simulink model "AXU5EV_Motor_Control_System"  (R2026b)
settings: Solver=FixedStepDiscrete  StopTime=0.1
model workspace (MAT data in the model file):
  ADC_Calibration_Log2_N = 10
  ADC_Manual_Offset_Valid_A = 0
  ADC_Manual_Offset_Valid_B = 0
  Angle_Init_EN = Simulink.Signal
  Angle_Init_EN.InitialValue = '0'
  Angle_Init_EN.DataType = 'double'
  Encoder_Counts_Per_Electrical_Period = 30000
  Encoder_Nanometres_Per_Count = 1000
  Experiment_Id_Limit_A = 0.5
  Experiment_Iq_Limit_A = 0.3
  Experiment_Parameter_Version = 20261117
  FOC_Fixed_Config.Version = 20261024
  FOC_Fixed_Config.Parameters.Rs = 1.45
  FOC_Fixed_Config.Parameters.Ld = 0.0118
  FOC_Fixed_Config.Parameters.Lq = 0.0118
  FOC_Fixed_Config.Parameters.psi = 0.0684240400279
  FOC_Fixed_Config.Parameters.Kp_ACR = 59
  FOC_Fixed_Config.Parameters.Ki_ACR = 7250
  FOC_Fixed_Config.Parameters.Kaw_d = 0.0122881355932
  FOC_Fixed_Config.Parameters.Kaw_q = 0.0122881355932
  FOC_Fixed_Config.Parameters.Ts_ACR = 0.0001
  FOC_Fixed_Config.Parameters.Udc = 48
  FOC_Fixed_Config.Fimath = embedded.fimath
  FOC_Fixed_Config.Fimath.RoundMode = 'convergent'
  FOC_Fixed_Config.Fimath.RoundingMethod = 'Convergent'
  FOC_Fixed_Config.Fimath.OverflowMode = 'saturate'
  FOC_Fixed_Config.Fimath.OverflowAction = 'Saturate'
  FOC_Fixed_Config.Fimath.ProductMode = 'FullPrecision'
  FOC_Fixed_Config.Fimath.SumMode = 'FullPrecision'
  FOC_Fixed_Config.Fimath.FixedOpFloatingYields = 'Fixed'
  FOC_Fixed_Config.Fimath.ProductWordLength = 32
  FOC_Fixed_Config.Fimath.SumWordLength = 32
  FOC_Fixed_Config.Fimath.MaxProductWordLength = 65535
  FOC_Fixed_Config.Fimath.MaxSumWordLength = 65535
  FOC_Fixed_Config.Fimath.ProductFractionLength = 30
  FOC_Fixed_Config.Fimath.ProductFixedExponent = -30
  FOC_Fixed_Config.Fimath.SumFractionLength = 30
  FOC_Fixed_Config.Fimath.SumFixedExponent = -30
  FOC_Fixed_Config.Fimath.SumSlopeAdjustmentFactor = 1
  FOC_Fixed_Config.Fimath.SumBias = 0
  FOC_Fixed_Config.Fimath.ProductSlopeAdjustmentFactor = 1
  FOC_Fixed_Config.Fimath.ProductBias = 0
  FOC_Fixed_Config.Fimath.CastBeforeSum = 1
  FOC_Fixed_Config.Fimath.SumSlope = 9.31322574615e-10
  FOC_Fixed_Config.Fimath.ProductSlope = 9.31322574615e-10
  FOC_Fixed_Config.Fimath.DDGMaxProductWordLength = 65535
  FOC_Fixed_Config.Fimath.DDGMaxSumWordLength = 65535
  FOC_Fixed_Config.Fimath.DDGProductFixedExponent = -30
  FOC_Fixed_Config.Fimath.DDGProductFractionLength = 30
  FOC_Fixed_Config.Fimath.DDGProductWordLength = 32
  FOC_Fixed_Config.Fimath.DDGSumFixedExponent = -30
  FOC_Fixed_Config.Fimath.DDGSumFractionLength = 30
  FOC_Fixed_Config.Fimath.DDGSumWordLength = 32
  FOC_Fixed_Config.Fimath.DDGProductBias = 0
  FOC_Fixed_Config.Fimath.DDGProductSlopeAdjustmentFactor = 1
  FOC_Fixed_Config.Fimath.DDGSumBias = 0
  FOC_Fixed_Config.Fimath.DDGSumSlopeAdjustmentFactor = 1
  FOC_Fixed_Config.Fimath.DDGCastBeforeSum = 1
  FOC_Fixed_Config.Fimath.DDGProductSlope = 9.31322574615e-10
  FOC_Fixed_Config.Fimath.DDGSumSlope = 9.31322574615e-10
  FOC_Fixed_Config.Types.Current = embedded.numerictype
  FOC_Fixed_Config.Types.Current.ReadOnly = 0
  FOC_Fixed_Config.Types.Current.Volatile = 0
  FOC_Fixed_Config.Types.Current.DataTypeMode = 'Fixed-point: binary point scaling'
  FOC_Fixed_Config.Types.Current.DataType = 'Fixed'
  FOC_Fixed_Config.Types.Current.Scaling = 'BinaryPoint'
  FOC_Fixed_Config.Types.Current.SignednessBool = 1
  FOC_Fixed_Config.Types.Current.Signedness = 'Signed'
  FOC_Fixed_Config.Types.Current.Signed = 1
  FOC_Fixed_Config.Types.Current.WordLength = 32
  FOC_Fixed_Config.Types.Current.FractionLength = 24
  FOC_Fixed_Config.Types.Current.BinaryPoint = 24
  FOC_Fixed_Config.Types.Current.Slope = 5.96046447754e-08
  FOC_Fixed_Config.Types.Current.FixedExponent = -24
  FOC_Fixed_Config.Types.Current.SlopeAdjustmentFactor = 1
  FOC_Fixed_Config.Types.Current.Bias = 0
  FOC_Fixed_Config.Types.Current.DataTypeOverride = 'Inherit'
  FOC_Fixed_Config.Types.Angle = embedded.numerictype
  FOC_Fixed_Config.Types.Angle.ReadOnly = 0
  FOC_Fixed_Config.Types.Angle.Volatile = 0
  FOC_Fixed_Config.Types.Angle.DataTypeMode = 'Fixed-point: binary point scaling'
  FOC_Fixed_Config.Types.Angle.DataType = 'Fixed'
  FOC_Fixed_Config.Types.Angle.Scaling = 'BinaryPoint'
  FOC_Fixed_Config.Types.Angle.SignednessBool = 1
  FOC_Fixed_Config.Types.Angle.Signedness = 'Signed'
  FOC_Fixed_Config.Types.Angle.Signed = 1
  FOC_Fixed_Config.Types.Angle.WordLength = 40
  FOC_Fixed_Config.Types.Angle.FractionLength = 32
  FOC_Fixed_Config.Types.Angle.BinaryPoint = 32
  FOC_Fixed_Config.Types.Angle.Slope = 2.32830643654e-10
  FOC_Fixed_Config.Types.Angle.FixedExponent = -32
  FOC_Fixed_Config.Types.Angle.SlopeAdjustmentFactor = 1
  FOC_Fixed_Config.Types.Angle.Bias = 0
  FOC_Fixed_Config.Types.Angle.DataTypeOverride = 'Inherit'
  FOC_Fixed_Config.Types.Omega = embedded.numerictype
  FOC_Fixed_Config.Types.Omega.ReadOnly = 0
  FOC_Fixed_Config.Types.Omega.Volatile = 0
  FOC_Fixed_Config.Types.Omega.DataTypeMode = 'Fixed-point: binary point scaling'
  FOC_Fixed_Config.Types.Omega.DataType = 'Fixed'
  FOC_Fixed_Config.Types.Omega.Scaling = 'BinaryPoint'
  FOC_Fixed_Config.Types.Omega.SignednessBool = 1
  FOC_Fixed_Config.Types.Omega.Signedness = 'Signed'
  FOC_Fixed_Config.Types.Omega.Signed = 1
  FOC_Fixed_Config.Types.Omega.WordLength = 40
  FOC_Fixed_Config.Types.Omega.FractionLength = 24
  FOC_Fixed_Config.Types.Omega.BinaryPoint = 24
  FOC_Fixed_Config.Types.Omega.Slope = 5.96046447754e-08
  FOC_Fixed_Config.Types.Omega.FixedExponent = -24
  FOC_Fixed_Config.Types.Omega.SlopeAdjustmentFactor = 1
  FOC_Fixed_Config.Types.Omega.Bias = 0
  FOC_Fixed_Config.Types.Omega.DataTypeOverride = 'Inherit'
  FOC_Fixed_Config.Types.Bus = embedded.numerictype
  FOC_Fixed_Config.Types.Bus.ReadOnly = 0
  FOC_Fixed_Config.Types.Bus.Volatile = 0
  FOC_Fixed_Config.Types.Bus.DataTypeMode = 'Fixed-point: binary point scaling'
  FOC_Fixed_Config.Types.Bus.DataType = 'Fixed'
  FOC_Fixed_Config.Types.Bus.Scaling = 'BinaryPoint'
  FOC_Fixed_Config.Types.Bus.SignednessBool = 0
  FOC_Fixed_Config.Types.Bus.Signedness = 'Unsigned'
  FOC_Fixed_Config.Types.Bus.Signed = 0
  FOC_Fixed_Config.Types.Bus.WordLength = 32
  FOC_Fixed_Config.Types.Bus.FractionLength = 24
  FOC_Fixed_Config.Types.Bus.BinaryPoint = 24
  FOC_Fixed_Config.Types.Bus.Slope = 5.96046447754e-08
  FOC_Fixed_Config.Types.Bus.FixedExponent = -24
  FOC_Fixed_Config.Types.Bus.SlopeAdjustmentFactor = 1
  FOC_Fixed_Config.Types.Bus.Bias = 0
  FOC_Fixed_Config.Types.Bus.DataTypeOverride = 'Inherit'
  FOC_Fixed_Config.Types.Work = embedded.numerictype
  FOC_Fixed_Config.Types.Work.ReadOnly = 0
  FOC_Fixed_Config.Types.Work.Volatile = 0
  FOC_Fixed_Config.Types.Work.DataTypeMode = 'Fixed-point: binary point scaling'
  FOC_Fixed_Config.Types.Work.DataType = 'Fixed'
  FOC_Fixed_Config.Types.Work.Scaling = 'BinaryPoint'
  FOC_Fixed_Config.Types.Work.SignednessBool = 1
  FOC_Fixed_Config.Types.Work.Signedness = 'Signed'
  FOC_Fixed_Config.Types.Work.Signed = 1
  FOC_Fixed_Config.Types.Work.WordLength = 64
  FOC_Fixed_Config.Types.Work.FractionLength = 40
  FOC_Fixed_Config.Types.Work.BinaryPoint = 40
  FOC_Fixed_Config.Types.Work.Slope = 9.09494701773e-13
  FOC_Fixed_Config.Types.Work.FixedExponent = -40
  FOC_Fixed_Config.Types.Work.SlopeAdjustmentFactor = 1
  FOC_Fixed_Config.Types.Work.Bias = 0
  FOC_Fixed_Config.Types.Work.DataTypeOverride = 'Inherit'
  FOC_Fixed_Config.Types.Square = embedded.numerictype
  FOC_Fixed_Config.Types.Square.ReadOnly = 0
  FOC_Fixed_Config.Types.Square.Volatile = 0
  FOC_Fixed_Config.Types.Square.DataTypeMode = 'Fixed-point: binary point scaling'
  FOC_Fixed_Config.Types.Square.DataType = 'Fixed'
  FOC_Fixed_Config.Types.Square.Scaling = 'BinaryPoint'
  FOC_Fixed_Config.Types.Square.SignednessBool = 0
  FOC_Fixed_Config.Types.Square.Signedness = 'Unsigned'
  FOC_Fixed_Config.Types.Square.Signed = 0
  FOC_Fixed_Config.Types.Square.WordLength = 64
  FOC_Fixed_Config.Types.Square.FractionLength = 36
  FOC_Fixed_Config.Types.Square.BinaryPoint = 36
  FOC_Fixed_Config.Types.Square.Slope = 1.45519152284e-11
  FOC_Fixed_Config.Types.Square.FixedExponent = -36
  FOC_Fixed_Config.Types.Square.SlopeAdjustmentFactor = 1
  FOC_Fixed_Config.Types.Square.Bias = 0
  FOC_Fixed_Config.Types.Square.DataTypeOverride = 'Inherit'
  FOC_Fixed_Config.Types.DivideWide = embedded.numerictype
  FOC_Fixed_Config.Types.DivideWide.ReadOnly = 0
  FOC_Fixed_Config.Types.DivideWide.Volatile = 0
  FOC_Fixed_Config.Types.DivideWide.DataTypeMode = 'Fixed-point: binary point scaling'
  FOC_Fixed_Config.Types.DivideWide.DataType = 'Fixed'
  FOC_Fixed_Config.Types.DivideWide.Scaling = 'BinaryPoint'
  FOC_Fixed_Config.Types.DivideWide.SignednessBool = 0
  FOC_Fixed_Config.Types.DivideWide.Signedness = 'Unsigned'
  FOC_Fixed_Config.Types.DivideWide.Signed = 0
  FOC_Fixed_Config.Types.DivideWide.WordLength = 72
  FOC_Fixed_Config.Types.DivideWide.FractionLength = 40
  FOC_Fixed_Config.Types.DivideWide.BinaryPoint = 40
  FOC_Fixed_Config.Types.DivideWide.Slope = 9.09494701773e-13
  FOC_Fixed_Config.Types.DivideWide.FixedExponent = -40
  FOC_Fixed_Config.Types.DivideWide.SlopeAdjustmentFactor = 1
  FOC_Fixed_Config.Types.DivideWide.Bias = 0
  FOC_Fixed_Config.Types.DivideWide.DataTypeOverride = 'Inherit'
  FOC_Fixed_Config.Types.Duty = embedded.numerictype
  FOC_Fixed_Config.Types.Duty.ReadOnly = 0
  FOC_Fixed_Config.Types.Duty.Volatile = 0
  FOC_Fixed_Config.Types.Duty.DataTypeMode = 'Fixed-point: binary point scaling'
  FOC_Fixed_Config.Types.Duty.DataType = 'Fixed'
  FOC_Fixed_Config.Types.Duty.Scaling = 'BinaryPoint'
  FOC_Fixed_Config.Types.Duty.SignednessBool = 0
  FOC_Fixed_Config.Types.Duty.Signedness = 'Unsigned'
  FOC_Fixed_Config.Types.Duty.Signed = 0
  FOC_Fixed_Config.Types.Duty.WordLength = 32
  FOC_Fixed_Config.Types.Duty.FractionLength = 30
  FOC_Fixed_Config.Types.Duty.BinaryPoint = 30
  FOC_Fixed_Config.Types.Duty.Slope = 9.31322574615e-10
  FOC_Fixed_Config.Types.Duty.FixedExponent = -30
  FOC_Fixed_Config.Types.Duty.SlopeAdjustmentFactor = 1
  FOC_Fixed_Config.Types.Duty.Bias = 0
  FOC_Fixed_Config.Types.Duty.DataTypeOverride = 'Inherit'
  FOC_Fixed_Config.Types.Coefficient = embedded.numerictype
  FOC_Fixed_Config.Types.Coefficient.ReadOnly = 0
  FOC_Fixed_Config.Types.Coefficient.Volatile = 0
  FOC_Fixed_Config.Types.Coefficient.DataTypeMode = 'Fixed-point: binary point scaling'
  FOC_Fixed_Config.Types.Coefficient.DataType = 'Fixed'
  FOC_Fixed_Config.Types.Coefficient.Scaling = 'BinaryPoint'
  FOC_Fixed_Config.Types.Coefficient.SignednessBool = 1
  FOC_Fixed_Config.Types.Coefficient.Signedness = 'Signed'
  FOC_Fixed_Config.Types.Coefficient.Signed = 1
  FOC_Fixed_Config.Types.Coefficient.WordLength = 64
  FOC_Fixed_Config.Types.Coefficient.FractionLength = 40
  FOC_Fixed_Config.Types.Coefficient.BinaryPoint = 40
  FOC_Fixed_Config.Types.Coefficient.Slope = 9.09494701773e-13
  FOC_Fixed_Config.Types.Coefficient.FixedExponent = -40
  FOC_Fixed_Config.Types.Coefficient.SlopeAdjustmentFactor = 1
  FOC_Fixed_Config.Types.Coefficient.Bias = 0
  FOC_Fixed_Config.Types.Coefficient.DataTypeOverride = 'Inherit'
  FOC_Fixed_Config.Types.Time = embedded.numerictype
  FOC_Fixed_Config.Types.Time.ReadOnly = 0
  FOC_Fixed_Config.Types.Time.Volatile = 0
  FOC_Fixed_Config.Types.Time.DataTypeMode = 'Fixed-point: binary point scaling'
  FOC_Fixed_Config.Types.Time.DataType = 'Fixed'
  FOC_Fixed_Config.Types.Time.Scaling = 'BinaryPoint'
  FOC_Fixed_Config.Types.Time.SignednessBool = 1
  FOC_Fixed_Config.Types.Time.Signedness = 'Signed'
  FOC_Fixed_Config.Types.Time.Signed = 1
  FOC_Fixed_Config.Types.Time.WordLength = 64
  FOC_Fixed_Config.Types.Time.FractionLength = 40
  FOC_Fixed_Config.Types.Time.BinaryPoint = 40
  FOC_Fixed_Config.Types.Time.Slope = 9.09494701773e-13
  FOC_Fixed_Config.Types.Time.FixedExponent = -40
  FOC_Fixed_Config.Types.Time.SlopeAdjustmentFactor = 1
  FOC_Fixed_Config.Types.Time.Bias = 0
  FOC_Fixed_Config.Types.Time.DataTypeOverride = 'Inherit'
  FOC_Fixed_Config.Types.Reset = 'boolean'
  FOC_Fixed_Config.Types.Sector = 'uint8'
  FOC_Fixed_Config.TypeStrings.Current = 'fixdt(1,32,24)'
  FOC_Fixed_Config.TypeStrings.Angle = 'fixdt(1,40,32)'
  FOC_Fixed_Config.TypeStrings.Omega = 'fixdt(1,40,24)'
  FOC_Fixed_Config.TypeStrings.Bus = 'fixdt(0,32,24)'
  FOC_Fixed_Config.TypeStrings.Work = 'fixdt(1,64,40)'
  FOC_Fixed_Config.TypeStrings.Square = 'fixdt(0,64,36)'
  FOC_Fixed_Config.TypeStrings.DivideWide = 'fixdt(0,72,40)'
  FOC_Fixed_Config.TypeStrings.Duty = 'fixdt(0,32,30)'
  FOC_Fixed_Config.TypeStrings.Coefficient = 'fixdt(1,64,40)'
  FOC_Fixed_Config.TypeStrings.Time = 'fixdt(1,64,40)'
  FOC_Fixed_Config.TypeStrings.Reset = 'boolean'
  FOC_Fixed_Config.TypeStrings.Sector = 'uint8'
  FOC_Fixed_Config.Ranges.phase_current_A = 2
  FOC_Fixed_Config.Ranges.reference_A = 2
  FOC_Fixed_Config.Ranges.theta_abs_rad = 25.1327412287
  FOC_Fixed_Config.Ranges.omega_abs_radps = 100
  FOC_Fixed_Config.Ranges.Vdc_min_V = 12
  FOC_Fixed_Config.Ranges.Vdc_max_V = 60
  FOC_Fixed_Config.Ranges.verified_duration_s = 60
  FOC_Fixed_Config.Ranges.state_initial_V = 0
  FOC_Fixed_Config.Ranges.scope = 'engineering verification envelope, not motor/drive ratings'
  FOC_Fixed_Config.Ranges.park_axis_bound_A = 3.52766841475
  FOC_Fixed_Config.Ranges.error_bound_A = 5.52766841475
  FOC_Fixed_Config.Ranges.feedforward_bound_V = 11.0050527322
  FOC_Fixed_Config.Ranges.integrator_bound_V = 703.086461988
  FOC_Fixed_Config.Ranges.raw_voltage_bound_V = 1040.22395119
  FOC_Fixed_Config.Ranges.square_sum_bound_V2 = 2164131.73726
  FOC_Fixed_Config.Coefficients.Kp.original = 59
  FOC_Fixed_Config.Coefficients.Kp.quantized = 59
  FOC_Fixed_Config.Coefficients.Kp.error = -1.42108547152e-14
  FOC_Fixed_Config.Coefficients.KiTs.original = 0.725
  FOC_Fixed_Config.Coefficients.KiTs.quantized = 0.725
  FOC_Fixed_Config.Coefficients.KiTs.error = 3.63709062867e-13
  FOC_Fixed_Config.Coefficients.Kaw_d.original = 0.0122881355932
  FOC_Fixed_Config.Coefficients.Kaw_d.quantized = 0.0122881355928
  FOC_Fixed_Config.Coefficients.Kaw_d.error = -3.94628774103e-13
  FOC_Fixed_Config.Coefficients.Kaw_q.original = 0.0122881355932
  FOC_Fixed_Config.Coefficients.Kaw_q.quantized = 0.0122881355928
  FOC_Fixed_Config.Coefficients.Kaw_q.error = -3.94628774103e-13
  FOC_Fixed_Config.Coefficients.Ld.original = 0.0118
  FOC_Fixed_Config.Coefficients.Ld.quantized = 0.0118000000002
  FOC_Fixed_Config.Coefficients.Ld.error = 2.21189386251e-13
  FOC_Fixed_Config.Coefficients.Lq.original = 0.0118
  FOC_Fixed_Config.Coefficients.Lq.quantized = 0.0118000000002
  FOC_Fixed_Config.Coefficients.Lq.error = 2.21189386251e-13
  FOC_Fixed_Config.Coefficients.psi.original = 0.0684240400279
  FOC_Fixed_Config.Coefficients.psi.quantized = 0.0684240400278
  FOC_Fixed_Config.Coefficients.psi.error = -1.18724474696e-13
  FOC_Fixed_Config.Coefficients.Ts.original = 0.0001
  FOC_Fixed_Config.Coefficients.Ts.quantized = 0.000100000000202
  FOC_Fixed_Config.Coefficients.Ts.error = 2.02271616882e-13
  FOC_Fixed_Config.Coefficients.InvSqrt3.original = 0.57735026919
  FOC_Fixed_Config.Coefficients.InvSqrt3.quantized = 0.57735026919
  FOC_Fixed_Config.Coefficients.InvSqrt3.error = 3.66262575824e-13
  FOC_Fixed_Config.Coefficients.TwoThird.original = 0.666666666667
  FOC_Fixed_Config.Coefficients.TwoThird.quantized = 0.666666666667
  FOC_Fixed_Config.Coefficients.TwoThird.error = 3.03201908025e-13
  FOC_Fixed_Config.Coefficients.C0866.original = 0.866
  FOC_Fixed_Config.Coefficients.C0866.quantized = 0.866
  FOC_Fixed_Config.Coefficients.C0866.error = -1.45439216226e-14
  FOC_Fixed_Config.Coefficients.C17321.original = 1.7321
  FOC_Fixed_Config.Coefficients.C17321.quantized = 1.7321
  FOC_Fixed_Config.Coefficients.C17321.error = 1.73194791842e-13
  FOC_Fixed_Config.Coefficients.C09.original = 0.9
  FOC_Fixed_Config.Coefficients.C09.quantized = 0.9
  FOC_Fixed_Config.Coefficients.C09.error = -3.6382008517e-13
  FOC_Fixed_Config.Coefficients.C0999.original = 0.999
  FOC_Fixed_Config.Coefficients.C0999.quantized = 0.999
  FOC_Fixed_Config.Coefficients.C0999.error = -2.03725925019e-13
  FOC_Fixed_Config.Coefficients.Epsilon.original = 1e-06
  FOC_Fixed_Config.Coefficients.Epsilon.quantized = 1.00000033854e-06
  FOC_Fixed_Config.Coefficients.Epsilon.error = 3.38535755918e-13
  FOC_Fixed_Config.Coefficients.DutyGain.original = -20000
  FOC_Fixed_Config.Coefficients.DutyGain.quantized = -20000
  FOC_Fixed_Config.Coefficients.DutyGain.error = 0
  FOC_Fixed_Parameters.Rs = 1.45
  FOC_Fixed_Parameters.Ld = 0.0118
  FOC_Fixed_Parameters.Lq = 0.0118
  FOC_Fixed_Parameters.psi = 0.0684240400279
  FOC_Fixed_Parameters.Kp_ACR = 59
  FOC_Fixed_Parameters.Ki_ACR = 7250
  FOC_Fixed_Parameters.Kaw_d = 0.0122881355932
  FOC_Fixed_Parameters.Kaw_q = 0.0122881355932
  FOC_Fixed_Parameters.Ts_ACR = 0.0001
  FOC_Fixed_Parameters.Udc = 48
  Feedback_Id_Step = 500
  Feedback_Tick_Hz = 50000000
  Feedback_Tick_Step = 5000
  Grating_Resolution_mm_per_count = 0.001
  Hardware_Binding_Complete = 0
  Hold_Ticks = 30000
  Host_AutoStart_EN = 0
  Host_Load_N = 0
  Host_Ready_Ticks = 5
  Host_Speed_Ramp_s = 0.2
  Host_Start_s = 0.05
  Host_Traj_Amax = 200
  Host_Traj_Jmax = 1000
  Host_Traj_Vmax = 20
  Id_Init_Step = 5e-05
  Id_Init_Target = 0.5
  Id_Release_Ramp_Ticks = 2000
  Init_Done = Simulink.Signal
  Init_Done.InitialValue = '0'
  Init_Done.DataType = 'double'
  Init_State_Num = Simulink.Signal
  Init_State_Num.InitialValue = '0'
  Init_State_Num.DataType = 'double'
  Iq_fric_run = 0.05
  Iq_fric_start = 0.4
  Iq_int_limit = 0.2
  Kaw_d = 0.0122881355932
  Kaw_q = 0.0122881355932
  Kaw_s = 0.4
  Ki_ACR = 7250
  Ki_ASR = 0.05
  Kp_ACR = 59
  Kp_ASR = 0.03
  Kp_pos = 5
  PMLSM_Kf_peak_N_per_Apeak = 21.4960461481
  PMLSM_Ld_H = 0.0118
  PMLSM_Lq_H = 0.0118
  PMLSM_Rs_ohm = 1.45
  PMLSM_psi_f_Wb = 0.0684240400279
  PMLSM_tau_NN_m = 0.03
  Physical_Calibration_Valid = 0
  Pos_deadband = 0.02
  Ramp_Ticks = 10000
  Speed_loop_Iq_Limit = 0.3
  Tau_e_mm = 30
  Theta_Offset_Fine = 0
  Theta_Offset_auto = Simulink.Signal
  Theta_Offset_auto.InitialValue = '0'
  Theta_Offset_auto.DataType = 'double'
  Total_Moving_Mass_Known = 0
  Total_Moving_Mass_kg = nan
  Ts = 0.0001
  Ts_ACR = 0.0001
  Ts_ASR = 0.001
  Ts_POS = 0.01
  Tuning_Current_Xi = 0.707106781187
  Udc = 48
  V_meas_max = 500
  V_pos_max_mmps = 20
  X_max_hard = 120
  X_max_soft = 110
  X_min_hard = -120
  X_min_soft = -110
  delay_N = 50
  id_init_ref = Simulink.Signal
  id_init_ref.InitialValue = '0'
  id_init_ref.DataType = 'double'
  theta_align_const = 0
  v_ff_eps = 0.5
  v_meas_zero_eps = 0.5
  v_over_eps = 3
  v_ref_max = 20
  v_ref_set_rate_dn = 100
  v_ref_set_rate_up = 100
  v_ref_set_step_dn = 0.01
  v_ref_set_step_up = 0.01
  v_ref_zero_eps = 0
  x_align_mm_latch = Simulink.Signal
  x_align_mm_latch.InitialValue = '0'
  x_align_mm_latch.DataType = 'double'
undefined symbols (not defined in the file): v_stick_off, v_stick_on
libraries: simulink x8
(part 1 of 2)
settings Model: Creator=lww  LastModifiedBy=lww
settings DataIOCC: SignalLogging=off
settings OptimizationCC: DefaultParameterBehavior=Inlined  DifferentSizesBufferReuse=on  EfficientTunableParamExpr=on  EnhancedBackFolding=on  OptimizationCustomize=off  OptimizeBlockOrder=speed  PassReuseOutputArgsAs=Individual arguments
settings DebuggingCC: ParameterTunabilityLossMsg=error
settings HardwareCC: ProdHWDeviceType=ARM Compatible->ARM Cortex-R  ProdLargestAtomicFloat=Double  ProdLargestAtomicInteger=Long  ProdLongLongMode=on
settings SFSimCC: MATLABDynamicMemAlloc=off
settings RTWCC: DataTypeReplacement=CDataTypesFixedWidth  Description=Embedded Coder  GenCodeOnly=on  SystemTargetFile=ert.tlc  TemplateMakefile=ert_default_tmf
settings CodeAppCC: ForceParamTrailComments=on  IgnoreCustomStorageClasses=off  InsertBlockDesc=on  OperatorAnnotations=on  SFDataObjDesc=on  SimulinkDataObjDesc=on
settings ERTTargetCC: CombineSignalStateStructs=on  GenerateSampleERTMain=on  MaxIdInt16=INT16_MAX  MaxIdInt32=INT32_MAX  MaxIdInt64=INT64_MAX  MaxIdInt8=INT8_MAX  MaxIdUint16=UINT16_MAX  MaxIdUint32=UINT32_MAX  MaxIdUint64=UINT64_MAX  MaxIdUint8=UINT8_MAX  MinIdInt16=INT16_MIN  MinIdInt32=INT32_MIN  MinIdInt64=INT64_MIN  MinIdInt8=INT8_MIN

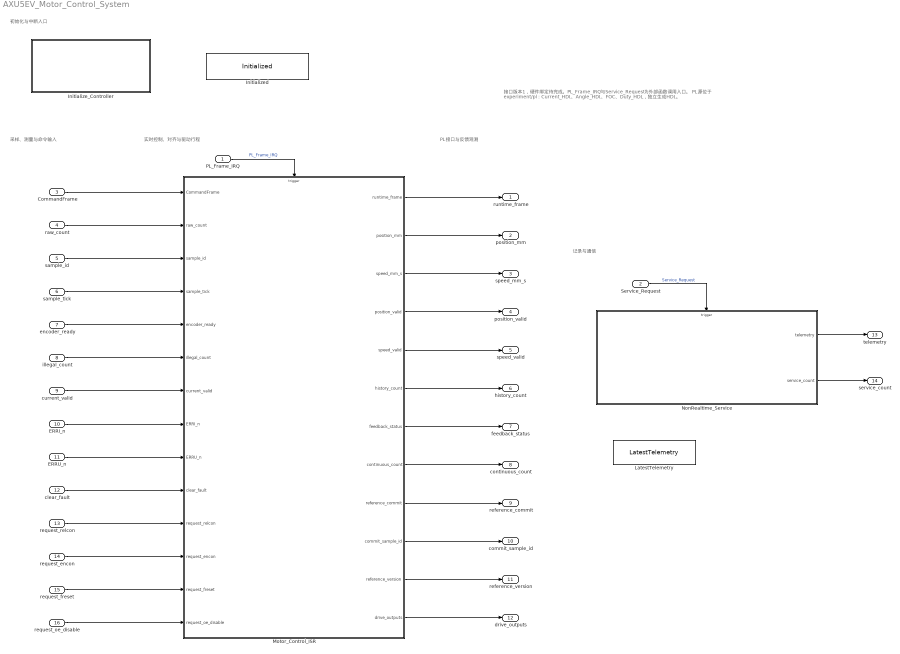
== system AXU5EV_Motor_Control_System ==
  note: 初始化与中断入口
  note: 采样、测量与命令输入
  note: 实时控制、对齐与驱动行程
  note: PL接口与反馈观测
  note: 记录与通信
  note: 接口版本1，硬件绑定待完成。PL_Frame_IRQ与Service_Request为外部函数调用入口。
      | PL源位于 experiment/pl：Current_HDL、Angle_HDL、FOC、Duty_HDL，独立生成HDL。
  PL_Frame_IRQ : Inport  Description=External function-call entry at each accepted 100us ADC/QEP feedback frame. HW_BINDING_PENDING: physical PL IRQ/GIC registration and atomic driver binding.  OutputFunctionCall=on
  Service_Request : Inport  Description=Externally scheduled non-real-time service. Copies latest 12-field telemetry and counts calls. IRQ preemption-consistent snapshot/communications binding pending in delivery B.  Port=2  OutputFunctionCall=on
  CommandFrame : Inport  Description=Interface version 1, 20 double internal fields. Binder overrides measured speed/position/fault and disables replay. See AX04 report for exact field groups.  Port=3  OutDataTypeStr=double  PortDimensions=20  Interpolate=off
  raw_count : Inport  Port=4  OutDataTypeStr=uint32  PortDimensions=1  Interpolate=off
  sample_id : Inport  Port=5  OutDataTypeStr=uint32  PortDimensions=1  Interpolate=off
  sample_tick : Inport  Description=uint64 timestamp in the existing 50MHz feedback clock domain, tick unit 20ns. Belongs to the same frozen frame as sample_id/raw_count.  Port=6  OutDataTypeStr=uint64  PortDimensions=1  Interpolate=off
  encoder_ready : Inport  Port=7  OutDataTypeStr=boolean  PortDimensions=1  Interpolate=off
  illegal_count : Inport  Port=8  OutDataTypeStr=uint32  PortDimensions=1  Interpolate=off
  current_valid : Inport  Port=9  OutDataTypeStr=boolean  PortDimensions=1  Interpolate=off
  ERRI_n : Inport  Port=10  OutDataTypeStr=boolean  PortDimensions=1  Interpolate=off
  ERRU_n : Inport  Port=11  OutDataTypeStr=boolean  PortDimensions=1  Interpolate=off
  clear_fault : Inport  Port=12  OutDataTypeStr=boolean  PortDimensions=1  Interpolate=off
  request_relcon : Inport  Port=13  OutDataTypeStr=boolean  PortDimensions=1  Interpolate=off
  request_encon : Inport  Port=14  OutDataTypeStr=boolean  PortDimensions=1  Interpolate=off
  request_freset : Inport  Port=15  OutDataTypeStr=boolean  PortDimensions=1  Interpolate=off
  request_oe_disable : Inport  Port=16  OutDataTypeStr=boolean  PortDimensions=1  Interpolate=off
  Initialize_Controller : Subsystem  TreatAsAtomicUnit=on
  Initialized : DataStoreMemory  DataStoreName=Initialized  WriteAfterWriteMsg=warning  InitialValue=false  ShowAdditionalParam=off  OutDataTypeStr=boolean  Dimensions=1
  LatestTelemetry : DataStoreMemory  DataStoreName=LatestTelemetry  WriteAfterWriteMsg=warning  InitialValue=zeros(12,1)  ShowAdditionalParam=off  OutDataTypeStr=double  Dimensions=12
  Motor_Control_ISR : Subsystem
  NonRealtime_Service : Subsystem  Description=Service_Request copies the latest 12-value telemetry and increments a software counter. Communication, long recording and preemption-consistent snapshots are HW_BINDING_PENDING.
  runtime_frame : Outport  OutDataTypeStr=double  PortDimensions=41
  position_mm : Outport  Port=2  OutDataTypeStr=double  PortDimensions=1
  speed_mm_s : Outport  Port=3  OutDataTypeStr=double  PortDimensions=1
  position_valid : Outport  Port=4  OutDataTypeStr=boolean  PortDimensions=1
  speed_valid : Outport  Port=5  OutDataTypeStr=boolean  PortDimensions=1
  history_count : Outport  Port=6  OutDataTypeStr=uint8  PortDimensions=1
  feedback_status : Outport  Description=PS feedback diagnostics. uint32 bits 0 startup, 1 duplicate, 2 missing frame, 3 configuration/history reset, 4 invalid encoder, 5 ambiguous half-wrap, 6 resynchronize.  Port=7  OutDataTypeStr=uint32  PortDimensions=1
  continuous_count : Outport  Port=8  OutDataTypeStr=int64  PortDimensions=1
  reference_commit : Outport  Description=PL command contract v1, 8 doubles. Id[A], Iq[A], omega[rad/s], offset[rad], alignment-angle bool, PWM permit bool, PI reset bool, valid bool.  Port=9  OutDataTypeStr=double  PortDimensions=8
  commit_sample_id : Outport  Port=10  OutDataTypeStr=uint32  PortDimensions=1
  reference_version : Outport  Port=11  OutDataTypeStr=uint32  PortDimensions=1
  drive_outputs : Outport  Description=PL/driver command contract v1, 5 bools. RELCON, ENCON, F_Reset, OE_disable, external fault latch. true OE_disable prohibits physical output. Hardware drivers pending.  Port=12  OutDataTypeStr=boolean  PortDimensions=5
  telemetry : Outport  Port=13  OutDataTypeStr=double  PortDimensions=12
  service_count : Outport  Port=14  OutDataTypeStr=uint32  PortDimensions=1
  wires:
  Motor_Control_ISR/12(drive_outputs) -> drive_outputs/1
  Motor_Control_ISR/11(reference_version) -> reference_version/1
  Motor_Control_ISR/10(commit_sample_id) -> commit_sample_id/1
  Motor_Control_ISR/9(reference_commit) -> reference_commit/1
  Motor_Control_ISR/8(continuous_count) -> continuous_count/1
  Motor_Control_ISR/7(feedback_status) -> feedback_status/1
  Motor_Control_ISR/6(history_count) -> history_count/1
  Motor_Control_ISR/5(speed_valid) -> speed_valid/1
  Motor_Control_ISR/4(position_valid) -> position_valid/1
  Motor_Control_ISR/3(speed_mm_s) -> speed_mm_s/1
  Motor_Control_ISR/2(position_mm) -> position_mm/1
  Motor_Control_ISR/1(runtime_frame) -> runtime_frame/1
  NonRealtime_Service/2(service_count) -> service_count/1
  NonRealtime_Service/1(telemetry) -> telemetry/1
  Service_Request/1 -> NonRealtime_Service/Trigger  "Service_Request"
  CommandFrame/1 -> Motor_Control_ISR/1(CommandFrame)
  raw_count/1 -> Motor_Control_ISR/2(raw_count)
  sample_id/1 -> Motor_Control_ISR/3(sample_id)
  sample_tick/1 -> Motor_Control_ISR/4(sample_tick)
  encoder_ready/1 -> Motor_Control_ISR/5(encoder_ready)
  illegal_count/1 -> Motor_Control_ISR/6(illegal_count)
  current_valid/1 -> Motor_Control_ISR/7(current_valid)
  ERRI_n/1 -> Motor_Control_ISR/8(ERRI_n)
  ERRU_n/1 -> Motor_Control_ISR/9(ERRU_n)
  clear_fault/1 -> Motor_Control_ISR/10(clear_fault)
  request_relcon/1 -> Motor_Control_ISR/11(request_relcon)
  request_encon/1 -> Motor_Control_ISR/12(request_encon)
  request_freset/1 -> Motor_Control_ISR/13(request_freset)
  request_oe_disable/1 -> Motor_Control_ISR/14(request_oe_disable)
  PL_Frame_IRQ/1 -> Motor_Control_ISR/Trigger  "PL_Frame_IRQ"

== system AXU5EV_Motor_Control_System/Initialize_Controller ==
  Event Listener : EventListener  DisableCoverage=on  EventName=reset
  Initialization_Complete : Constant  Value=true  OutDataTypeStr=boolean
  Set_Controller_Initialized : DataStoreWrite  DataStoreName=Initialized  IndexOptions=Index vector (dialog)  Indices=1  OutputSizes=1
  wires:
  Initialization_Complete/1 -> Set_Controller_Initialized/1

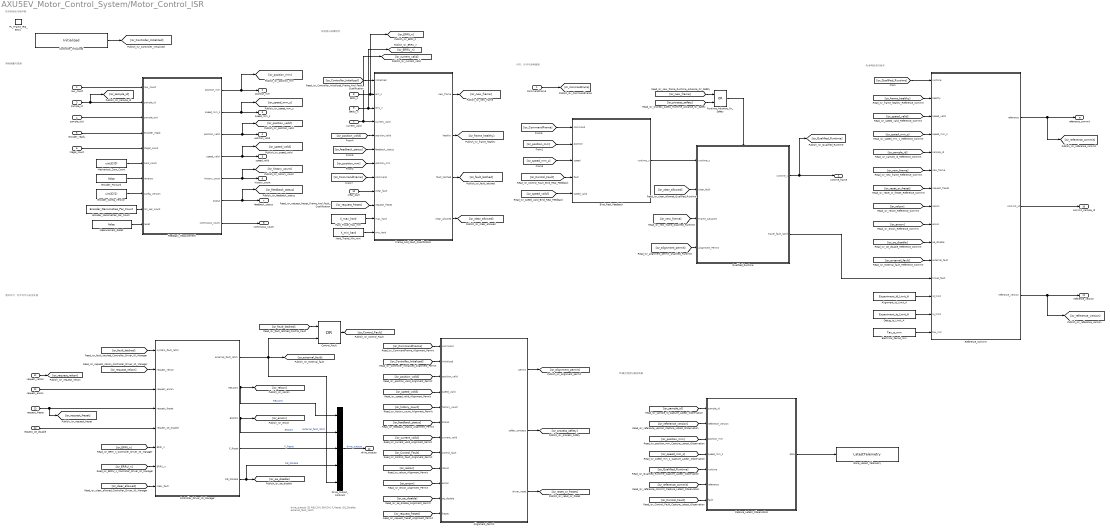
== system AXU5EV_Motor_Control_System/Motor_Control_ISR ==
  note: 软件初始化与帧中断
  note: 同帧测量与观测
  note: 对齐、外环与参考管理
  note: 驱动许可、对齐许可与安全处理
  note: PL参考封装与版本
  note: PS最近观测与服务数据
  note: 帧资格与故障锁存
  note: drive_outputs [5]
      | RELCON, ENCON, F_Reset, OE_Disable, external_fault_latch
  CommandFrame : Inport  OutDataTypeStr=double  PortDimensions=20  Interpolate=off
  raw_count : Inport  Port=2  OutDataTypeStr=uint32  PortDimensions=1  Interpolate=off
  sample_id : Inport  Port=3  OutDataTypeStr=uint32  PortDimensions=1  Interpolate=off
  sample_tick : Inport  Port=4  OutDataTypeStr=uint64  PortDimensions=1  Interpolate=off
  encoder_ready : Inport  Port=5  OutDataTypeStr=boolean  PortDimensions=1  Interpolate=off
  illegal_count : Inport  Port=6  OutDataTypeStr=uint32  PortDimensions=1  Interpolate=off
  current_valid : Inport  Port=7  OutDataTypeStr=boolean  PortDimensions=1  Interpolate=off
  ERRI_n : Inport  Port=8  OutDataTypeStr=boolean  PortDimensions=1  Interpolate=off
  ERRU_n : Inport  Port=9  OutDataTypeStr=boolean  PortDimensions=1  Interpolate=off
  clear_fault : Inport  Port=10  OutDataTypeStr=boolean  PortDimensions=1  Interpolate=off
  request_relcon : Inport  Port=11  OutDataTypeStr=boolean  PortDimensions=1  Interpolate=off
  request_encon : Inport  Port=12  OutDataTypeStr=boolean  PortDimensions=1  Interpolate=off
  request_freset : Inport  Port=13  OutDataTypeStr=boolean  PortDimensions=1  Interpolate=off
  request_oe_disable : Inport  Port=14  OutDataTypeStr=boolean  PortDimensions=1  Interpolate=off
  PL_Frame_IRQ_Entry : TriggerPort  TriggerType=function-call  VariantControl=(inherit)  PortDimensions=1
  Alignment_Id_Limit_A : Constant  Value=Experiment_Id_Limit_A  OutDataTypeStr=double
  Alignment_Permit : MATLAB Function  TreatAsAtomicUnit=on
  Bind_Real_Feedback : Subsystem
  Capture_Latest_Observation : MATLAB Function  TreatAsAtomicUnit=on
  Control_Fault : Logic  Operator=OR  IconShape=distinctive  AllPortsSameDT=off  OutDataTypeStr=boolean
  Controller_Driver_IO_Manager : Subsystem  Description=Use-site driver logic consumes the upper system_fault latch and active-low ERRI_n/ERRU_n. F_Reset inhibits REL/EN and stays distinct from qualified software clear. Physical fast inhibit and output level bindings remain pending.
  Controller_Initialized : DataStoreRead  Description=Initialized records software initialization only. Physical feedback, current establishment and hardware binding are separate.  DataStoreName=Initialized  IndexOptions=Index vector (dialog)  Indices=1  OutputSizes=1
  Debug_Iq_Limit_A : Constant  Value=Experiment_Iq_Limit_A  OutDataTypeStr=double
  Drive_Output_Contract : Mux  Inputs=5
  Electrical_Period_mm : Constant  Value=Tau_e_mm  OutDataTypeStr=double
  Encoder_Config_Version : Constant  Value=uint32(1)  OutDataTypeStr=uint32
  Encoder_Forward : Constant  Value=false  OutDataTypeStr=boolean
  Encoder_Nanometres_Per_Count : Constant  Value=Encoder_Nanometres_Per_Count  OutDataTypeStr=uint32
  Feedback_Measurement : Subsystem  Description=DSP Caculate_measurement SID465 + count-origin SID1055 and Gain5 SID1058. Reused Delay50/Add1/Gain1. Qualified 100us history, 50 intervals=5ms, 51 observations before valid speed. No IIR. nm_per_count, zero and direction remain explicit inputs. Duplicate frames hold history.
  Frame_And_Fault_Qualification : MATLAB Function  TreatAsAtomicUnit=on
  Hard_Travel_Max_mm : Constant  Value=X_max_hard  OutDataTypeStr=double
  Hard_Travel_Min_mm : Constant  Value=X_min_hard  OutDataTypeStr=double
  Measurement_Reset : Constant  Value=false  OutDataTypeStr=boolean
  Mechanical_Zero_Count : Constant  Value=uint32(0)  OutDataTypeStr=uint32
  Qualified_Runtime : Subsystem
  Reference_Commit : MATLAB Function  Description=Packages Id[A], Iq[A], omega[rad/s], offset[rad], alignment angle selection, PWM permit, PI reset and reference valid plus frame/version. HW_BINDING_PENDING for atomic AXI submission.  TreatAsAtomicUnit=on
  Runtime_Advance_Or_Safety : Logic  Operator=OR  AllPortsSameDT=off  OutDataTypeStr=boolean
  Store_Latest_Telemetry : DataStoreWrite  DataStoreName=LatestTelemetry  IndexOptions=Index vector (dialog)  Indices=1  OutputSizes=1
  runtime_frame : Outport  OutDataTypeStr=double  PortDimensions=41
  position_mm : Outport  Port=2  OutDataTypeStr=double  PortDimensions=1
  speed_mm_s : Outport  Port=3  OutDataTypeStr=double  PortDimensions=1
  position_valid : Outport  Port=4  OutDataTypeStr=boolean  PortDimensions=1
  speed_valid : Outport  Port=5  OutDataTypeStr=boolean  PortDimensions=1
  history_count : Outport  Port=6  OutDataTypeStr=uint8  PortDimensions=1
  feedback_status : Outport  Port=7  OutDataTypeStr=uint32  PortDimensions=1
  continuous_count : Outport  Port=8  OutDataTypeStr=int64  PortDimensions=1
  reference_commit : Outport  Port=9  OutDataTypeStr=double  PortDimensions=8  InitialOutput=[0;0;0;0;0;0;1;0]
  commit_sample_id : Outport  Port=10  OutDataTypeStr=uint32  PortDimensions=1
  reference_version : Outport  Port=11  OutDataTypeStr=uint32  PortDimensions=1
  drive_outputs : Outport  Port=12  OutDataTypeStr=boolean  PortDimensions=5  InitialOutput=[false;false;false;true;false]
  wires:
  [isr_CommandFrame] -> Alignment_Permit/1(command)
  [isr_Controller_Initialized] -> Alignment_Permit/2(initialized)
  [isr_position_valid] -> Alignment_Permit/3(position_valid)
  [isr_speed_valid] -> Alignment_Permit/4(speed_valid)
  [isr_history_count] -> Alignment_Permit/5(history_count)
  [isr_feedback_status] -> Alignment_Permit/6(status)
  [isr_current_valid] -> Alignment_Permit/7(current_valid)
  [isr_Control_Fault] -> Alignment_Permit/8(control_fault)
  [isr_relcon] -> Alignment_Permit/9(relcon)
  [isr_encon] -> Alignment_Permit/10(encon)
  [isr_oe_disable] -> Alignment_Permit/11(oe_disable)
  [isr_request_freset] -> Alignment_Permit/12(freset)
  CommandFrame/1 -> [isr_CommandFrame]
  Feedback_Measurement/1(position_mm) -> position_mm/1, [isr_position_mm]
  Feedback_Measurement/2(speed_mm_s) -> speed_mm_s/1, [isr_speed_mm_s]
  [isr_Control_Fault] -> Bind_Real_Feedback/4(fault)
  Feedback_Measurement/4(speed_valid) -> [isr_speed_valid], speed_valid/1
  [isr_sample_id] -> Capture_Latest_Observation/1(sample_id)
  [isr_reference_version] -> Capture_Latest_Observation/2(reference_version)
  [isr_position_mm] -> Capture_Latest_Observation/3(position_mm)
  [isr_speed_mm_s] -> Capture_Latest_Observation/4(speed_mm_s)
  [isr_Qualified_Runtime] -> Capture_Latest_Observation/5(runtime)
  [isr_reference_commit] -> Capture_Latest_Observation/6(reference)
  [isr_Control_Fault] -> Capture_Latest_Observation/7(fault)
  [isr_fault_latched] -> Control_Fault/1
  Controller_Driver_IO_Manager/1(external_fault_latch) -> [isr_external_fault], Drive_Output_Contract/5, Control_Fault/2  "external_fault_latch"
  [isr_fault_latched] -> Controller_Driver_IO_Manager/1(system_fault_latch)
  [isr_request_relcon] -> Controller_Driver_IO_Manager/2(request_relcon)
  request_encon/1 -> Controller_Driver_IO_Manager/3(request_encon)
  request_freset/1 -> Controller_Driver_IO_Manager/4(request_freset), [isr_request_freset]
  request_oe_disable/1 -> Controller_Driver_IO_Manager/5(request_oe_disable)
  [isr_ERRI_n] -> Controller_Driver_IO_Manager/6(ERRI_n)
  [isr_ERRU_n] -> Controller_Driver_IO_Manager/7(ERRU_n)
  [isr_clear_allowed] -> Controller_Driver_IO_Manager/8(clear_fault)
  Controller_Driver_IO_Manager/2(RELCON) -> Drive_Output_Contract/1, [isr_relcon]  "RELCON"
  Controller_Driver_IO_Manager/3(ENCON) -> Drive_Output_Contract/2, [isr_encon]  "ENCON"
  Controller_Driver_IO_Manager/4(F_Reset) -> Drive_Output_Contract/3  "F_Reset"
  Controller_Driver_IO_Manager/5(OE_Disable) -> Drive_Output_Contract/4, [isr_oe_disable]  "OE_Disable"
  raw_count/1 -> Feedback_Measurement/1(raw_count)
  sample_id/1 -> Feedback_Measurement/2(sample_id), [isr_sample_id]
  sample_tick/1 -> Feedback_Measurement/3(sample_tick)
  encoder_ready/1 -> Feedback_Measurement/4(encoder_ready)
  illegal_count/1 -> Feedback_Measurement/5(illegal_count)
  Mechanical_Zero_Count/1 -> Feedback_Measurement/6(zero_count)
  Encoder_Forward/1 -> Feedback_Measurement/7(reverse)
  Encoder_Config_Version/1 -> Feedback_Measurement/8(config_version)
  Encoder_Nanometres_Per_Count/1 -> Feedback_Measurement/9(nm_per_count)
  Measurement_Reset/1 -> Feedback_Measurement/10(reset)
  [isr_Controller_Initialized] -> Frame_And_Fault_Qualification/1(initialized)
  ERRI_n/1 -> Frame_And_Fault_Qualification/2(erri_n), [isr_ERRI_n]
  ERRU_n/1 -> Frame_And_Fault_Qualification/3(erru_n), [isr_ERRU_n]
  current_valid/1 -> Frame_And_Fault_Qualification/4(current_valid), [isr_current_valid]
  Feedback_Measurement/3(position_valid) -> [isr_position_valid], position_valid/1
  Feedback_Measurement/6(status) -> feedback_status/1, [isr_feedback_status]
  clear_fault/1 -> Frame_And_Fault_Qualification/9(clear_fault)
  [isr_request_freset] -> Frame_And_Fault_Qualification/10(request_freset)
  Hard_Travel_Max_mm/1 -> Frame_And_Fault_Qualification/11(max_hard)
  Hard_Travel_Min_mm/1 -> Frame_And_Fault_Qualification/12(min_hard)
  Control_Fault/1 -> [isr_Control_Fault]
  Controller_Initialized/1 -> [isr_Controller_Initialized]
  Qualified_Runtime/1(runtime_y) -> [isr_Qualified_Runtime], runtime_frame/1
  Alignment_Permit/1(permit) -> [isr_alignment_permit]
  Frame_And_Fault_Qualification/4(clear_allowed) -> [isr_clear_allowed]
  Frame_And_Fault_Qualification/3(fault_latched) -> [isr_fault_latched]
  Frame_And_Fault_Qualification/2(healthy) -> [isr_frame_healthy]
  Feedback_Measurement/5(history_count) -> [isr_history_count], history_count/1
  Frame_And_Fault_Qualification/1(new_frame) -> [isr_new_frame]
  Alignment_Permit/2(safety_process) -> [isr_process_safety]
  Reference_Commit/1(reference) -> [isr_reference_commit], reference_commit/1
  Reference_Commit/3(reference_version) -> [isr_reference_version], reference_version/1
  request_relcon/1 -> [isr_request_relcon]
  Alignment_Permit/3(driver_reset) -> [isr_reset_or_freset]
  Runtime_Advance_Or_Safety/1 -> Qualified_Runtime/Enable
  Bind_Real_Feedback/1(runtime_u) -> Qualified_Runtime/1(runtime_u)
  [isr_clear_allowed] -> Qualified_Runtime/2(clear_fault)
  [isr_new_frame] -> Qualified_Runtime/3(Frame_Advance)
  [isr_alignment_permit] -> Qualified_Runtime/4(Alignment_Permit)
  [isr_frame_healthy] -> Reference_Commit/2(healthy)
  [isr_speed_valid] -> Reference_Commit/3(speed_valid)
  [isr_speed_mm_s] -> Reference_Commit/4(speed_mm_s)
  [isr_sample_id] -> Reference_Commit/5(sample_id)
  [isr_new_frame] -> Reference_Commit/6(new_frame)
  [isr_reset_or_freset] -> Reference_Commit/7(request_freset)
  [isr_relcon] -> Reference_Commit/8(relcon)
  [isr_encon] -> Reference_Commit/9(encon)
  [isr_oe_disable] -> Reference_Commit/10(oe_disable)
  [isr_external_fault] -> Reference_Commit/11(external_fault)
  Qualified_Runtime/2(travel_fault_latch) -> Reference_Commit/12(travel_fault)
  Alignment_Id_Limit_A/1 -> Reference_Commit/13(id_limit)
  Debug_Iq_Limit_A/1 -> Reference_Commit/14(iq_limit)
  Electrical_Period_mm/1 -> Reference_Commit/15(tau_mm)
  [isr_new_frame] -> Runtime_Advance_Or_Safety/1
  [isr_process_safety] -> Runtime_Advance_Or_Safety/2
  Capture_Latest_Observation/1(data) -> Store_Latest_Telemetry/1
  Feedback_Measurement/7(continuous_count) -> continuous_count/1
  Reference_Commit/2(commit_id) -> commit_sample_id/1
  Drive_Output_Contract/1 -> drive_outputs/1  "drive_outputs"
  [isr_Qualified_Runtime] -> Reference_Commit/1(runtime)
  [isr_position_mm] -> Bind_Real_Feedback/2(position)
  [isr_position_mm] -> Frame_And_Fault_Qualification/7(position_mm)
  [isr_speed_mm_s] -> Bind_Real_Feedback/3(speed)
  [isr_position_valid] -> Frame_And_Fault_Qualification/5(position_valid)
  [isr_feedback_status] -> Frame_And_Fault_Qualification/6(feedback_status)
  [isr_CommandFrame] -> Bind_Real_Feedback/1(command)
  [isr_CommandFrame] -> Frame_And_Fault_Qualification/8(command)
  [isr_speed_valid] -> Bind_Real_Feedback/5(speed_valid)

== system AXU5EV_Motor_Control_System/NonRealtime_Service ==
  Service_Entry : TriggerPort  TriggerType=function-call  VariantControl=(inherit)  PortDimensions=1
  Count_Service_Call : MATLAB Function  TreatAsAtomicUnit=on
  Read_Latest_Telemetry : DataStoreRead  DataStoreName=LatestTelemetry  IndexOptions=Index vector (dialog)  Indices=1  OutputSizes=1
  Service_Count_State : UnitDelay  InitialCondition=uint32(0)  SampleTime=-1
  telemetry : Outport  OutDataTypeStr=double  PortDimensions=12
  service_count : Outport  Port=2  OutDataTypeStr=uint32  PortDimensions=1
  wires:
  Count_Service_Call/1(next) -> Service_Count_State/1, service_count/1
  Service_Count_State/1 -> Count_Service_Call/1(previous)
  Read_Latest_Telemetry/1 -> telemetry/1

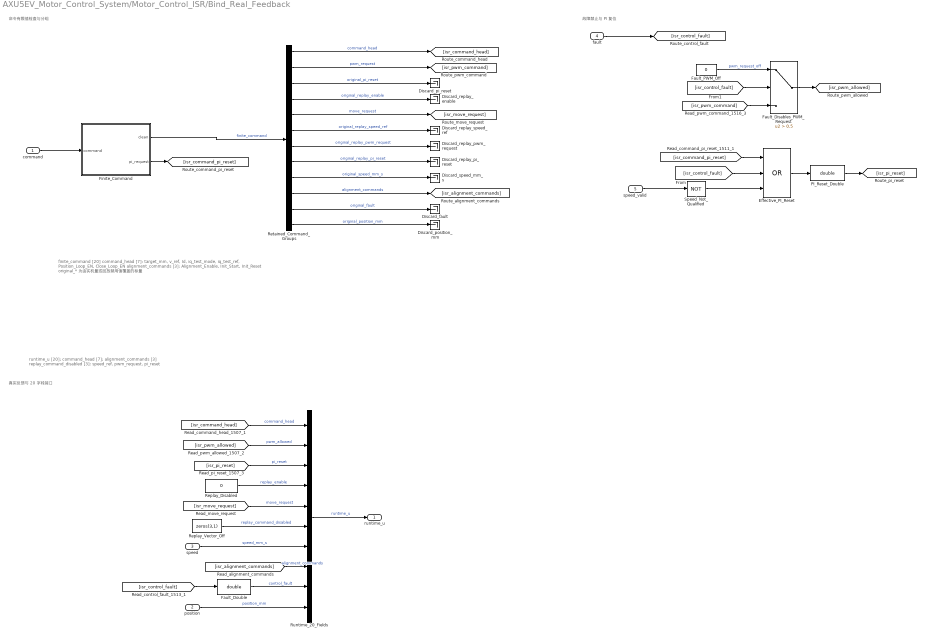
== system AXU5EV_Motor_Control_System/Motor_Control_ISR/Bind_Real_Feedback ==
  note: 命令有限值检查与分组
  note: 故障禁止与 PI 复位
  note: 真实反馈与 20 字段接口
  note: finite_command [20]
      | command_head [7]: target_mm, v_ref, Id, iq_test_mode, iq_test_ref, Position_Loop_EN, Close_Loop_EN
      | alignment_commands [3]: Alignment_Enable, Init_Start, Init_Reset
      | original_* 为由实机量或回放禁用值覆盖的标量
  note: runtime_u [20]; command_head [7]; alignment_commands [3]
      | replay_command_disabled [3]: speed_ref, pwm_request, pi_reset
  command : Inport  OutDataTypeStr=double
  position : Inport  Port=2  OutDataTypeStr=double
  speed : Inport  Port=3  OutDataTypeStr=double
  fault : Inport  Port=4  OutDataTypeStr=boolean
  speed_valid : Inport  Port=5  OutDataTypeStr=boolean
  Discard_fault : Terminator
  Discard_pi_reset : Terminator
  Discard_position_mm : Terminator
  Discard_replay_enable : Terminator
  Discard_replay_pi_reset : Terminator
  Discard_replay_pwm_request : Terminator
  Discard_replay_speed_ref : Terminator
  Discard_speed_mm_s : Terminator
  Effective_PI_Reset : Logic  Operator=OR  Inputs=3  IconShape=distinctive  AllPortsSameDT=off  OutDataTypeStr=boolean
  Fault_Disables_PWM_Request : Switch  Criteria=u2 > Threshold  Threshold=0.5  SaturateOnIntegerOverflow=off  InputSameDT=off
  Fault_Double : DataTypeConversion  OutDataTypeStr=double  SaturateOnIntegerOverflow=off  RndMeth=Floor
  Fault_PWM_Off : Constant  Value=0  OutDataTypeStr=double
  Finite_Command : MATLAB Function  TreatAsAtomicUnit=on
  PI_Reset_Double : DataTypeConversion  OutDataTypeStr=double  SaturateOnIntegerOverflow=off  RndMeth=Floor
  Replay_Disabled : Constant  Value=0  OutDataTypeStr=double
  Replay_Vector_Off : Constant  Value=zeros(3,1)
  Retained_Command_Groups : Demux  Outputs=[7 1 1 1 1 1 1 1 1 3 1 1]
  Runtime_20_Fields : Mux  Inputs=10
  Speed_Not_Qualified : Logic  Operator=NOT  IconShape=distinctive  AllPortsSameDT=off  OutDataTypeStr=boolean
  runtime_u : Outport  PortDimensions=20
  wires:
  speed_valid/1 -> Speed_Not_Qualified/1
  [isr_command_pi_reset] -> Effective_PI_Reset/1
  [isr_control_fault] -> Fault_Double/1
  [isr_command_head] -> Runtime_20_Fields/1  "command_head"
  [isr_pwm_allowed] -> Runtime_20_Fields/2  "pwm_allowed"
  [isr_pi_reset] -> Runtime_20_Fields/3  "pi_reset"
  [isr_move_request] -> Runtime_20_Fields/5  "move_request"
  [isr_alignment_commands] -> Runtime_20_Fields/8  "alignment_commands"
  [isr_pwm_command] -> Fault_Disables_PWM_Request/3
  command/1 -> Finite_Command/1(command)
  Finite_Command/1(clean) -> Retained_Command_Groups/1  "finite_command"
  Finite_Command/2(pi_request) -> [isr_command_pi_reset]
  fault/1 -> [isr_control_fault]
  Speed_Not_Qualified/1 -> Effective_PI_Reset/3
  Effective_PI_Reset/1 -> PI_Reset_Double/1
  Retained_Command_Groups/1 -> [isr_command_head]  "command_head"
  Fault_Disables_PWM_Request/1 -> [isr_pwm_allowed]
  PI_Reset_Double/1 -> [isr_pi_reset]
  Retained_Command_Groups/5 -> [isr_move_request]  "move_request"
  Replay_Vector_Off/1 -> Runtime_20_Fields/6  "replay_command_disabled"
  speed/1 -> Runtime_20_Fields/7  "speed_mm_s"
  Fault_Double/1 -> Runtime_20_Fields/9  "control_fault"
  position/1 -> Runtime_20_Fields/10  "position_mm"
  Retained_Command_Groups/2 -> [isr_pwm_command]  "pwm_request"
  Runtime_20_Fields/1 -> runtime_u/1  "runtime_u"
  [isr_control_fault] -> Effective_PI_Reset/2
  [isr_control_fault] -> Fault_Disables_PWM_Request/2
  Retained_Command_Groups/12 -> Discard_position_mm/1  "original_position_mm"
  Retained_Command_Groups/11 -> Discard_fault/1  "original_fault"
  Retained_Command_Groups/9 -> Discard_speed_mm_s/1  "original_speed_mm_s"
  Retained_Command_Groups/8 -> Discard_replay_pi_reset/1  "original_replay_pi_reset"
  Retained_Command_Groups/7 -> Discard_replay_pwm_request/1  "original_replay_pwm_request"
  Retained_Command_Groups/6 -> Discard_replay_speed_ref/1  "original_replay_speed_ref"
  Retained_Command_Groups/4 -> Discard_replay_enable/1  "original_replay_enable"
  Retained_Command_Groups/3 -> Discard_pi_reset/1  "original_pi_reset"
  Replay_Disabled/1 -> Runtime_20_Fields/4  "replay_enable"
  Fault_PWM_Off/1 -> Fault_Disables_PWM_Request/1  "pwm_request_off"
  Retained_Command_Groups/10 -> [isr_alignment_commands]  "alignment_commands"

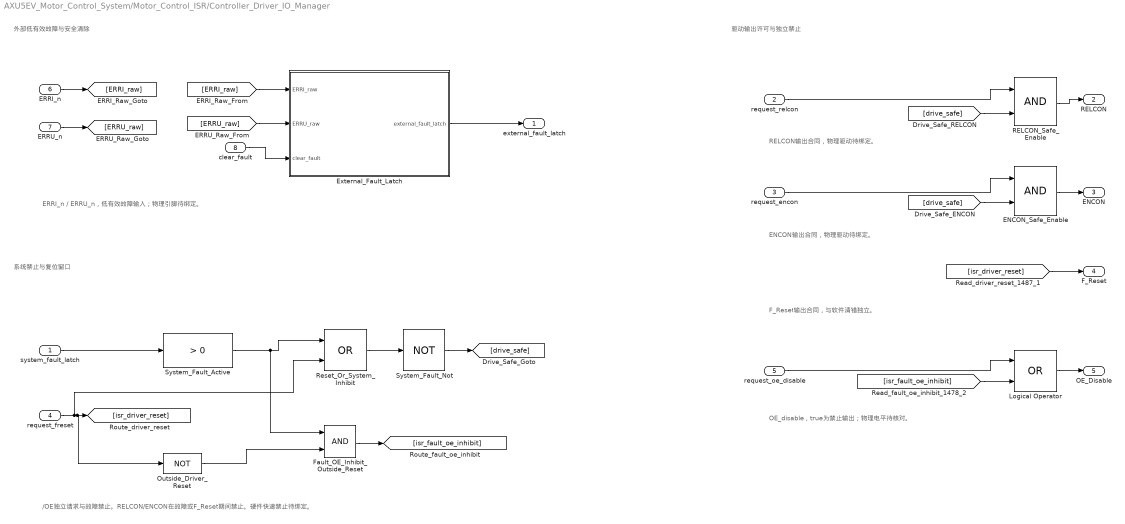
== system AXU5EV_Motor_Control_System/Motor_Control_ISR/Controller_Driver_IO_Manager ==
  note: 驱动输出许可与独立禁止
  note: 系统禁止与复位窗口
  note: 外部低有效故障与安全清除
  note: /OE独立请求与故障禁止。RELCON/ENCON在故障或F_Reset期间禁止。硬件快速禁止待绑定。
  note: ERRI_n / ERRU_n，低有效故障输入；物理引脚待绑定。
  note: RELCON输出合同，物理驱动待绑定。
  note: ENCON输出合同，物理驱动待绑定。
  note: F_Reset输出合同，与软件清错独立。
  note: OE_disable，true为禁止输出；物理电平待核对。
  system_fault_latch : Inport  OutDataTypeStr=boolean  PortDimensions=1
  request_relcon : Inport  Port=2  OutDataTypeStr=boolean  PortDimensions=1  Interpolate=off
  request_encon : Inport  Port=3  OutDataTypeStr=boolean  PortDimensions=1  Interpolate=off
  request_freset : Inport  Port=4  OutDataTypeStr=boolean  PortDimensions=1  Interpolate=off
  request_oe_disable : Inport  Port=5  OutDataTypeStr=boolean  PortDimensions=1  Interpolate=off
  ERRI_n : Inport  Port=6  OutDataTypeStr=boolean  PortDimensions=1  Interpolate=off
  ERRU_n : Inport  Port=7  OutDataTypeStr=boolean  PortDimensions=1  Interpolate=off
  clear_fault : Inport  Port=8  OutDataTypeStr=boolean  PortDimensions=1  Interpolate=off
  ENCON_Safe_Enable : Logic
  External_Fault_Latch : Subsystem
  Fault_OE_Inhibit_Outside_Reset : Logic  AllPortsSameDT=off  OutDataTypeStr=boolean
  Logical Operator : Logic  Operator=OR  AllPortsSameDT=off  OutDataTypeStr=boolean
  Outside_Driver_Reset : Logic  Operator=NOT  Inputs=1  AllPortsSameDT=off  OutDataTypeStr=boolean
  RELCON_Safe_Enable : Logic
  Reset_Or_System_Inhibit : Logic  Operator=OR  AllPortsSameDT=off  OutDataTypeStr=boolean
  System_Fault_Active : simulink/Logic and Bit Operations/Compare To Constant  relop=>  const=0  OutDataTypeStr=boolean
  System_Fault_Not : Logic  Operator=NOT  Inputs=1
  external_fault_latch : Outport  OutDataTypeStr=boolean  PortDimensions=1
  RELCON : Outport  Port=2  OutDataTypeStr=boolean  PortDimensions=1
  ENCON : Outport  Port=3  OutDataTypeStr=boolean  PortDimensions=1
  F_Reset : Outport  Port=4  OutDataTypeStr=boolean  PortDimensions=1
  OE_Disable : Outport  Port=5  OutDataTypeStr=boolean  PortDimensions=1
  wires:
  clear_fault/1 -> External_Fault_Latch/3(clear_fault)
  [ERRU_raw] -> External_Fault_Latch/2(ERRU_raw)
  ERRU_n/1 -> [ERRU_raw]
  ERRI_n/1 -> [ERRI_raw]
  [isr_fault_oe_inhibit] -> Logical Operator/2
  [isr_driver_reset] -> F_Reset/1
  System_Fault_Not/1 -> [drive_safe]
  request_encon/1 -> ENCON_Safe_Enable/1
  [drive_safe] -> ENCON_Safe_Enable/2
  [ERRI_raw] -> External_Fault_Latch/1(ERRI_raw)
  System_Fault_Active/1 -> Fault_OE_Inhibit_Outside_Reset/1, Reset_Or_System_Inhibit/1
  Outside_Driver_Reset/1 -> Fault_OE_Inhibit_Outside_Reset/2
  request_oe_disable/1 -> Logical Operator/1
  Fault_OE_Inhibit_Outside_Reset/1 -> [isr_fault_oe_inhibit]
  request_freset/1 -> Outside_Driver_Reset/1, [isr_driver_reset], Reset_Or_System_Inhibit/2
  request_relcon/1 -> RELCON_Safe_Enable/1
  [drive_safe] -> RELCON_Safe_Enable/2
  system_fault_latch/1 -> System_Fault_Active/1
  Reset_Or_System_Inhibit/1 -> System_Fault_Not/1
  External_Fault_Latch/1(external_fault_latch) -> external_fault_latch/1
  RELCON_Safe_Enable/1 -> RELCON/1
  ENCON_Safe_Enable/1 -> ENCON/1
  Logical Operator/1 -> OE_Disable/1

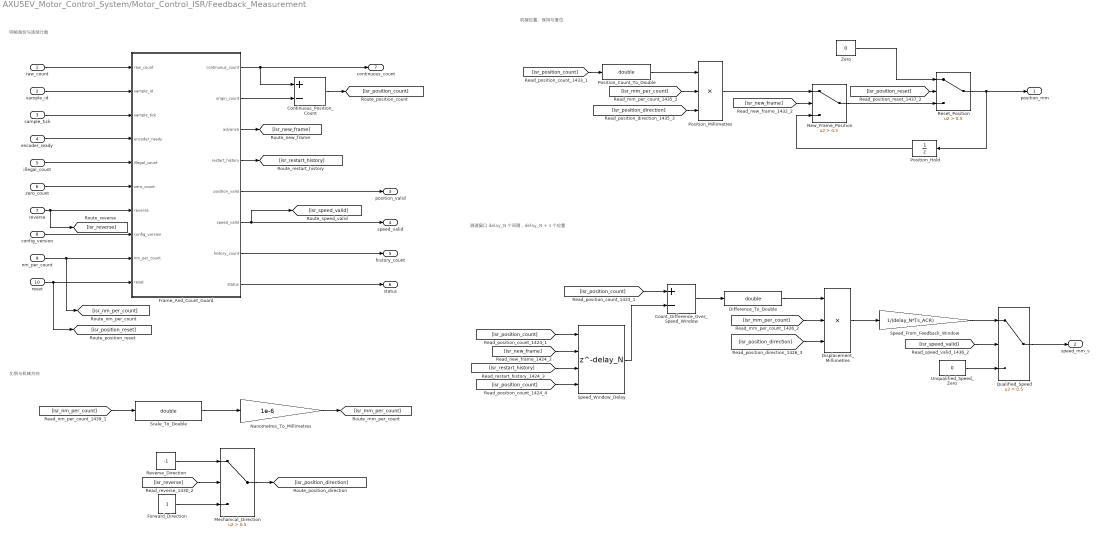
== system AXU5EV_Motor_Control_System/Motor_Control_ISR/Feedback_Measurement ==
  note: 同帧身份与连续计数
  note: 机械位置、保持与复位
  note: 测速窗口 delay_N 个间隔，delay_N + 1 个位置
  note: 比例与机械方向
  raw_count : Inport  OutDataTypeStr=uint32
  sample_id : Inport  Port=2  OutDataTypeStr=uint32
  sample_tick : Inport  Port=3  OutDataTypeStr=uint64
  encoder_ready : Inport  Port=4  OutDataTypeStr=boolean
  illegal_count : Inport  Port=5  OutDataTypeStr=uint32
  zero_count : Inport  Port=6  OutDataTypeStr=uint32
  reverse : Inport  Port=7  OutDataTypeStr=boolean
  config_version : Inport  Port=8  OutDataTypeStr=uint32
  nm_per_count : Inport  Port=9  OutDataTypeStr=uint32
  reset : Inport  Port=10  OutDataTypeStr=boolean
  Continuous_Position_Count : Sum  Inputs=+-  OutDataTypeStr=int64  AccumDataTypeStr=int64
  Count_Difference_Over_Speed_Window : Sum  Inputs=+-  OutDataTypeStr=int64  AccumDataTypeStr=int64
  Difference_To_Double : DataTypeConversion  OutDataTypeStr=double  SaturateOnIntegerOverflow=off  RndMeth=Floor
  Displacement_Millimetres : Product  Inputs=***  OutDataTypeStr=double
  Forward_Direction : Constant  OutDataTypeStr=double
  Frame_And_Count_Guard : MATLAB Function  TreatAsAtomicUnit=on
  Mechanical_Direction : Switch  Criteria=u2 > Threshold  Threshold=0.5  SaturateOnIntegerOverflow=off  InputSameDT=off
  Nanometres_To_Millimetres : Gain  Gain=1e-6  OutDataTypeStr=double
  New_Frame_Position : Switch  Criteria=u2 > Threshold  Threshold=0.5  SaturateOnIntegerOverflow=off  InputSameDT=off
  Position_Count_To_Double : DataTypeConversion  OutDataTypeStr=double  SaturateOnIntegerOverflow=off  RndMeth=Floor
  Position_Hold : UnitDelay  SampleTime=-1
  Position_Millimetres : Product  Inputs=***  OutDataTypeStr=double
  Qualified_Speed : Switch  Criteria=u2 > Threshold  Threshold=0.5  SaturateOnIntegerOverflow=off  InputSameDT=off
  Reset_Position : Switch  Criteria=u2 > Threshold  Threshold=0.5  SaturateOnIntegerOverflow=off  InputSameDT=off
  Reverse_Direction : Constant  Value=-1  OutDataTypeStr=double
  Scale_To_Double : DataTypeConversion  OutDataTypeStr=double  SaturateOnIntegerOverflow=off  RndMeth=Floor
  Speed_From_Feedback_Window : Gain  Gain=1/(delay_N*Ts_ACR)  OutDataTypeStr=double
  Speed_Window_Delay : Delay  DelayLength=delay_N  InitialConditionSource=Input port  ExternalReset=Level hold  ShowEnablePort=on
      settings: InputPortMap=u0,e6,r5,p4
  Unqualified_Speed_Zero : Constant  Value=0  OutDataTypeStr=double
  Zero : Constant  Value=0  OutDataTypeStr=double
  position_mm : Outport  OutDataTypeStr=double
  speed_mm_s : Outport  Port=2  OutDataTypeStr=double
  position_valid : Outport  Port=3  OutDataTypeStr=boolean
  speed_valid : Outport  Port=4  OutDataTypeStr=boolean
  history_count : Outport  Port=5  OutDataTypeStr=uint8
  status : Outport  Port=6  OutDataTypeStr=uint32
  continuous_count : Outport  Port=7  OutDataTypeStr=int64
  wires:
  raw_count/1 -> Frame_And_Count_Guard/1(raw_count)
  sample_id/1 -> Frame_And_Count_Guard/2(sample_id)
  sample_tick/1 -> Frame_And_Count_Guard/3(sample_tick)
  illegal_count/1 -> Frame_And_Count_Guard/5(illegal_count)
  Qualified_Speed/1 -> speed_mm_s/1
  [isr_position_reset] -> Reset_Position/2
  [isr_reverse] -> Mechanical_Direction/2
  [isr_new_frame] -> New_Frame_Position/2
  Frame_And_Count_Guard/8(status) -> status/1
  Frame_And_Count_Guard/7(history_count) -> history_count/1
  Frame_And_Count_Guard/5(position_valid) -> position_valid/1
  New_Frame_Position/1 -> Reset_Position/3
  Frame_And_Count_Guard/6(speed_valid) -> [isr_speed_valid], speed_valid/1
  Speed_From_Feedback_Window/1 -> Qualified_Speed/1
  Scale_To_Double/1 -> Nanometres_To_Millimetres/1
  Forward_Direction/1 -> Mechanical_Direction/3
  reset/1 -> [isr_position_reset], Frame_And_Count_Guard/10(reset)
  nm_per_count/1 -> Frame_And_Count_Guard/9(nm_per_count), [isr_nm_per_count]
  config_version/1 -> Frame_And_Count_Guard/8(config_version)
  reverse/1 -> [isr_reverse], Frame_And_Count_Guard/7(reverse)
  zero_count/1 -> Frame_And_Count_Guard/6(zero_count)
  encoder_ready/1 -> Frame_And_Count_Guard/4(encoder_ready)
  Mechanical_Direction/1 -> [isr_position_direction]
  Nanometres_To_Millimetres/1 -> [isr_mm_per_count]
  Frame_And_Count_Guard/4(restart_history) -> [isr_restart_history]
  Frame_And_Count_Guard/3(advance) -> [isr_new_frame]
  Continuous_Position_Count/1 -> [isr_position_count]
  Frame_And_Count_Guard/2(origin_count) -> Continuous_Position_Count/2
  Frame_And_Count_Guard/1(continuous_count) -> continuous_count/1, Continuous_Position_Count/1
  Unqualified_Speed_Zero/1 -> Qualified_Speed/3
  Speed_Window_Delay/1 -> Count_Difference_Over_Speed_Window/2
  Count_Difference_Over_Speed_Window/1 -> Difference_To_Double/1
  Displacement_Millimetres/1 -> Speed_From_Feedback_Window/1
  Reverse_Direction/1 -> Mechanical_Direction/1
  Position_Millimetres/1 -> New_Frame_Position/1
  Position_Hold/1 -> New_Frame_Position/3
  Reset_Position/1 -> position_mm/1, Position_Hold/1
  Position_Count_To_Double/1 -> Position_Millimetres/1
  Zero/1 -> Reset_Position/1
  [isr_position_count] -> Count_Difference_Over_Speed_Window/1
  [isr_position_count] -> Speed_Window_Delay/1
  [isr_position_count] -> Speed_Window_Delay/4
  [isr_position_count] -> Position_Count_To_Double/1
  [isr_new_frame] -> Speed_Window_Delay/2
  [isr_restart_history] -> Speed_Window_Delay/3
  [isr_mm_per_count] -> Displacement_Millimetres/2
  [isr_mm_per_count] -> Position_Millimetres/2
  [isr_position_direction] -> Displacement_Millimetres/3
  [isr_position_direction] -> Position_Millimetres/3
  [isr_nm_per_count] -> Scale_To_Double/1
  [isr_speed_valid] -> Qualified_Speed/2
  Difference_To_Double/1 -> Displacement_Millimetres/1

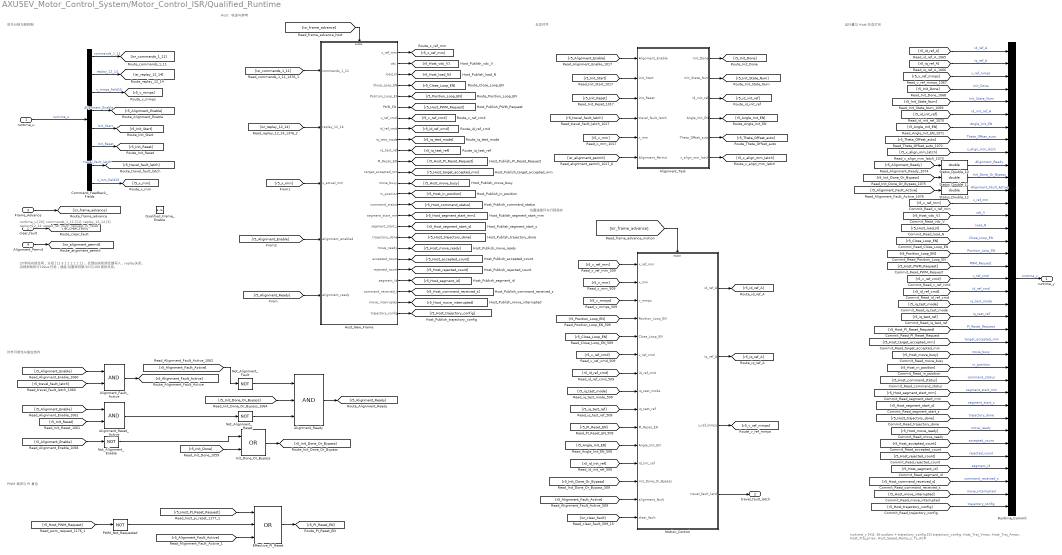
== system AXU5EV_Motor_Control_System/Motor_Control_ISR/Qualified_Runtime ==
  note: Host、轨迹与参考
  note: 五态对齐
  note: 位置速度环与行程保护
  note: 运行量与 Host 状态打包
  note: 20字段内部合同，分组 [11 3 1 1 1 1 1 1]。反馈由实机绑定器写入，replay关闭。
      | 合格新帧执行100us任务；速度/位置保持原/10与/100首拍关系。
  note: 命令分组与帧控制
  note: 对齐可用性与复位条件
  note: PWM 请求与 PI 复位
  note: runtime_u [20]; commands_1_11 [11]; replay_12_14 [3]
      | replay_12_14: speed_ref, pwm_request, pi_reset
  note: runtime_y [41]: 36 scalars + trajectory_config [5]
      | trajectory_config: Host_Traj_Vmax, Host_Traj_Amax, Host_Traj_Jmax, Host_Speed_Ramp_s, Ts_ACR
  runtime_u : Inport  PortDimensions=20
  clear_fault : Inport  Port=2  OutDataTypeStr=boolean  PortDimensions=1
  Frame_Advance : Inport  Port=3  OutDataTypeStr=boolean
  Alignment_Permit : Inport  Port=4  OutDataTypeStr=boolean
  Qualified_Frame_Enable : EnablePort
  Alignment_Fault_Active : Logic  IconShape=distinctive  AllPortsSameDT=off  OutDataTypeStr=boolean
  Alignment_Ready : Logic  Inputs=3  IconShape=distinctive  AllPortsSameDT=off  OutDataTypeStr=boolean
  Alignment_Reset_Active : Logic  IconShape=distinctive  AllPortsSameDT=off  OutDataTypeStr=boolean
  Alignment_Task : Subsystem
  Command_Feedback_Fields : Demux  Description=runtime_u（20字段）：1:11命令，12:14 replay[速度mm/s PWM PI_Reset]，15速度mm/s，16对齐使能，17 Start，18 Init_Reset，19行程故障，20位置mm。分组宽度=[11 3 1 1 1 1 1 1]。  Outputs=[11 3 1 1 1 1 1 1]
  Effective_PI_Reset : Logic  Operator=OR  Inputs=3  AllPortsSameDT=off  OutDataTypeStr=boolean
  Host_New_Frame : Subsystem
  Init_Done_Or_Bypass : Logic  Operator=OR  IconShape=distinctive  AllPortsSameDT=off  OutDataTypeStr=boolean
  Motion_Control : Subsystem
  Not_Alignment_Enable : Logic  Operator=NOT  IconShape=distinctive  AllPortsSameDT=off  OutDataTypeStr=boolean
  Not_Alignment_Fault : Logic  Operator=NOT  IconShape=distinctive  AllPortsSameDT=off  OutDataTypeStr=boolean
  Not_Alignment_Reset : Logic  Operator=NOT  IconShape=distinctive  AllPortsSameDT=off  OutDataTypeStr=boolean
  PWM_Not_Requested : Logic  Operator=NOT  AllPortsSameDT=off  OutDataTypeStr=boolean
  Runtime_Commit : Mux  Inputs=37
  Status_Double_10 : DataTypeConversion  OutDataTypeStr=double  SaturateOnIntegerOverflow=off  RndMeth=Floor
  Status_Double_11 : DataTypeConversion  OutDataTypeStr=double  SaturateOnIntegerOverflow=off  RndMeth=Floor
  Status_Double_12 : DataTypeConversion  OutDataTypeStr=double  SaturateOnIntegerOverflow=off  RndMeth=Floor
  runtime_y : Outport
  travel_fault_latch : Outport  Port=2  OutDataTypeStr=double  PortDimensions=1
  wires:
  [r5_x_ref_mm] -> Runtime_Commit/13  "x_ref_mm"
  [r5_v_ref_cmd] -> Runtime_Commit/19  "v_ref_cmd"
  [r5_Position_Loop_EN] -> Runtime_Commit/17  "Position_Loop_EN"
  [r5_Host_PWM_Request] -> Runtime_Commit/18  "PWM_Request"
  [r5_id_ref_cmd] -> Runtime_Commit/20  "id_ref_cmd"
  Status_Double_10/1 -> Runtime_Commit/10  "Alignment_Ready"
  [r5_Close_Loop_EN] -> Runtime_Commit/16  "Close_Loop_EN"
  [r5_Host_vdc_V] -> Runtime_Commit/14  "vdc_V"
  Status_Double_12/1 -> Runtime_Commit/12  "Alignment_Fault_Active"
  Status_Double_11/1 -> Runtime_Commit/11  "Init_Done_Or_Bypass"
  [r5_Host_trajectory_done] -> Runtime_Commit/30  "trajectory_done"
  Alignment_Reset_Active/1 -> Not_Alignment_Reset/1
  [r5_Host_load_N] -> Runtime_Commit/15  "load_N"
  [r5_Host_command_received_s] -> Runtime_Commit/35  "command_received_s"
  [r5_iq_test_mode] -> Runtime_Commit/21  "iq_test_mode"
  [r5_Position_Loop_EN] -> Motion_Control/4(Position_Loop_EN)
  [r5_iq_test_ref] -> Runtime_Commit/22  "iq_test_ref"
  [r5_Host_PI_Reset_Request] -> Runtime_Commit/23  "PI_Reset_Request"
  [r5_x_ref_mm] -> Motion_Control/1(x_ref_mm)
  [r5_Host_target_accepted_mm] -> Runtime_Commit/24  "target_accepted_mm"
  [r5_x_mm] -> Motion_Control/2(x_mm)
  [r5_Host_move_busy] -> Runtime_Commit/25  "move_busy"
  Motion_Control/1(id_ref_A) -> [r5_id_ref_A]
  [r5_v_mmps] -> Motion_Control/3(v_mmps)
  [r5_Host_in_position] -> Runtime_Commit/26  "in_position"
  [r5_Host_command_status] -> Runtime_Commit/27  "command_status"
  [r5_id_ref_cmd] -> Motion_Control/7(id_ref_cmd)
  [r5_Host_segment_start_s] -> Runtime_Commit/29  "segment_start_s"
  [r5_iq_test_mode] -> Motion_Control/8(iq_test_mode)
  [r5_iq_test_ref] -> Motion_Control/9(iq_test_ref)
  [r5_PI_Reset_EN] -> Motion_Control/10(PI_Reset_EN)
  [r5_Host_move_ready] -> Runtime_Commit/31  "move_ready"
  [r5_Angle_Init_EN] -> Motion_Control/11(Angle_Init_EN)
  [r5_id_init_ref] -> Motion_Control/12(id_init_ref)
  Motion_Control/3(v_ref_mmps) -> [r5_v_ref_mmps]
  [r5_Host_rejected_count] -> Runtime_Commit/33  "rejected_count"
  [r5_Init_Done_Or_Bypass] -> Motion_Control/13(Init_Done_Or_Bypass)
  [r5_travel_fault_latch] -> Alignment_Fault_Active/2
  [r5_Host_segment_id] -> Runtime_Commit/34  "segment_id"
  [r5_Alignment_Enable] -> Alignment_Fault_Active/1
  [r5_Alignment_Fault_Active] -> Motion_Control/14(alignment_fault)
  [r5_Alignment_Enable] -> Not_Alignment_Enable/1
  [r5_Host_move_interrupted] -> Runtime_Commit/36  "move_interrupted"
  [r5_Host_trajectory_config] -> Runtime_Commit/37  "trajectory_config"
  Motion_Control/4(travel_fault_latch) -> travel_fault_latch/1
  Command_Feedback_Fields/8 -> [r5_x_mm]  "x_mm_field20"
  Command_Feedback_Fields/7 -> [r5_travel_fault_latch]  "travel_fault_latch"
  Command_Feedback_Fields/5 -> [r5_Init_Start]  "Init_Start"
  Command_Feedback_Fields/4 -> [r5_Alignment_Enable]  "Alignment_Enable"
  Command_Feedback_Fields/6 -> [r5_Init_Reset]  "Init_Reset"
  runtime_u/1 -> Command_Feedback_Fields/1  "runtime_u"
  Command_Feedback_Fields/3 -> [r5_v_mmps]  "v_mmps_field15"
  Host_New_Frame/6(PWM_EN) -> [r5_Host_PWM_Request]
  Host_New_Frame/11(PI_Reset_EN) -> [r5_Host_PI_Reset_Request]
  [r5_x_mm] -> Host_New_Frame/3(x_actual_mm)
  [r5_Alignment_Enable] -> Host_New_Frame/4(alignment_enabled)
  [r5_Alignment_Ready] -> Host_New_Frame/5(alignment_ready)
  Host_New_Frame/1(x_ref_mm) -> [r5_x_ref_mm]
  Host_New_Frame/2(vdc) -> [r5_Host_vdc_V]
  Host_New_Frame/3(load_N) -> [r5_Host_load_N]
  Host_New_Frame/4(Close_Loop_EN) -> [r5_Close_Loop_EN]
  Host_New_Frame/5(Position_Loop_EN) -> [r5_Position_Loop_EN]
  Host_New_Frame/7(v_ref_cmd) -> [r5_v_ref_cmd]
  Host_New_Frame/8(id_ref_cmd) -> [r5_id_ref_cmd]
  Host_New_Frame/9(iq_test_mode) -> [r5_iq_test_mode]
  Host_New_Frame/10(iq_test_ref) -> [r5_iq_test_ref]
  Host_New_Frame/12(target_accepted_mm) -> [r5_Host_target_accepted_mm]
  Host_New_Frame/13(move_busy) -> [r5_Host_move_busy]
  Host_New_Frame/14(in_position) -> [r5_Host_in_position]
  Host_New_Frame/15(command_status) -> [r5_Host_command_status]
  Host_New_Frame/16(segment_start_mm) -> [r5_Host_segment_start_mm]
  Host_New_Frame/17(segment_start_s) -> [r5_Host_segment_start_s]
  Host_New_Frame/18(trajectory_done) -> [r5_Host_trajectory_done]
  Host_New_Frame/19(move_ready) -> [r5_Host_move_ready]
  Host_New_Frame/20(accepted_count) -> [r5_Host_accepted_count]
  Host_New_Frame/21(rejected_count) -> [r5_Host_rejected_count]
  Host_New_Frame/22(segment_id) -> [r5_Host_segment_id]
  Host_New_Frame/23(command_received_s) -> [r5_Host_command_received_s]
  Host_New_Frame/24(move_interrupted) -> [r5_Host_move_interrupted]
  Host_New_Frame/25(trajectory_config) -> [r5_Host_trajectory_config]
  [r5_Init_Reset] -> Alignment_Reset_Active/2
  Not_Alignment_Reset/1 -> Alignment_Ready/3
  [r5_Alignment_Enable] -> Alignment_Reset_Active/1
  [r5_Init_Done_Or_Bypass] -> Alignment_Ready/2
  Not_Alignment_Enable/1 -> Init_Done_Or_Bypass/1
  Alignment_Fault_Active/1 -> [r5_Alignment_Fault_Active]
  [r5_Alignment_Fault_Active] -> Not_Alignment_Fault/1
  Not_Alignment_Fault/1 -> Alignment_Ready/1
  [r5_v_ref_cmd] -> Motion_Control/6(v_ref_cmd)
  Alignment_Task/5(Theta_Offset_auto) -> [r5_Theta_Offset_auto]
  Alignment_Task/2(Init_State_Num) -> [r5_Init_State_Num]
  [r5_x_mm] -> Alignment_Task/5(x_mm)
  [r5_Init_Done_Or_Bypass] -> Status_Double_11/1
  [r5_Alignment_Fault_Active] -> Status_Double_12/1
  [r5_Alignment_Ready] -> Status_Double_10/1
  Alignment_Task/3(id_init_ref) -> [r5_id_init_ref]
  Init_Done_Or_Bypass/1 -> [r5_Init_Done_Or_Bypass]
  [r5_Init_Start] -> Alignment_Task/2(Init_Start)
  [r5_id_init_ref] -> Runtime_Commit/6  "id_init_ref_A"
  [r5_Init_Done] -> Init_Done_Or_Bypass/2
  [r5_travel_fault_latch] -> Alignment_Task/4(travel_fault_latch)
  [r5_Init_State_Num] -> Runtime_Commit/5  "Init_State_Num"
  [r5_Init_Done] -> Runtime_Commit/4  "Init_Done"
  Alignment_Ready/1 -> [r5_Alignment_Ready]
  [r5_Init_Reset] -> Alignment_Task/3(Init_Reset)
  Alignment_Task/1(Init_Done) -> [r5_Init_Done]
  [r5_x_align_mm_latch] -> Runtime_Commit/9  "x_align_mm_latch"
  [r5_Angle_Init_EN] -> Runtime_Commit/7  "Angle_Init_EN"
  [r5_iq_ref_A] -> Runtime_Commit/2  "iq_ref_A"
  [r5_v_ref_mmps] -> Runtime_Commit/3  "v_ref_mmps"
  [r5_id_ref_A] -> Runtime_Commit/1  "id_ref_A"
  Alignment_Task/6(x_align_mm_latch) -> [r5_x_align_mm_latch]
  [r5_Theta_Offset_auto] -> Runtime_Commit/8  "Theta_Offset_auto"
  [isr_clear_fault] -> Motion_Control/15(clear_fault)
  [isr_replay_12_14] -> Host_New_Frame/2(replay_12_14)
  [isr_commands_1_11] -> Host_New_Frame/1(commands_1_11)
  [r5_Host_PI_Reset_Request] -> Effective_PI_Reset/1
  [r5_Host_PWM_Request] -> PWM_Not_Requested/1
  [isr_alignment_permit] -> Alignment_Task/6(Alignment_Permit)
  [r5_Alignment_Enable] -> Alignment_Task/1(Alignment_Enable)
  Alignment_Task/4(Angle_Init_EN) -> [r5_Angle_Init_EN]
  [r5_Close_Loop_EN] -> Motion_Control/5(Close_Loop_EN)
  [r5_Host_segment_start_mm] -> Runtime_Commit/28  "segment_start_mm"
  Motion_Control/2(iq_ref_A) -> [r5_iq_ref_A]
  [r5_Host_accepted_count] -> Runtime_Commit/32  "accepted_count"
  clear_fault/1 -> [isr_clear_fault]
  Command_Feedback_Fields/2 -> [isr_replay_12_14]  "replay_12_14"
  Command_Feedback_Fields/1 -> [isr_commands_1_11]  "commands_1_11"
  PWM_Not_Requested/1 -> Effective_PI_Reset/2
  Alignment_Permit/1 -> [isr_alignment_permit]
  [r5_Alignment_Fault_Active] -> Effective_PI_Reset/3
  Effective_PI_Reset/1 -> [r5_PI_Reset_EN]
  Runtime_Commit/1 -> runtime_y/1  "runtime_y"
  [isr_frame_advance] -> Host_New_Frame/Enable
  [isr_frame_advance] -> Motion_Control/Enable
  Frame_Advance/1 -> [isr_frame_advance]

== system AXU5EV_Motor_Control_System/Motor_Control_ISR/Controller_Driver_IO_Manager/External_Fault_Latch ==
  note: 低有效输入与安全清除
  note: 故障置位与锁存回读
  ERRI_raw : Inport  OutDataTypeStr=boolean  PortDimensions=1
  ERRU_raw : Inport  Port=2  OutDataTypeStr=boolean  PortDimensions=1
  clear_fault : Inport  Port=3  OutDataTypeStr=boolean  PortDimensions=1  Interpolate=off
  Clear_Only_When_Raw_Healthy : Logic  Inputs=3  IconShape=distinctive  AllPortsSameDT=off  OutDataTypeStr=boolean
  ERRI_Active_Low : Logic  Operator=NOT  IconShape=distinctive
  ERRU_Active_Low : Logic  Operator=NOT  IconShape=distinctive
  External_Fault_Latch_OR : Logic  Operator=OR  IconShape=distinctive
  External_Fault_Latch_Z : UnitDelay  InitialCondition=false  SampleTime=-1
  External_Fault_OR : Logic  Operator=OR  IconShape=distinctive
  Retain_Unless_Safe_Clear : Logic  Operator=NOT  Inputs=1  IconShape=distinctive  AllPortsSameDT=off  OutDataTypeStr=boolean
  Retained_External_Fault : Logic  IconShape=distinctive  AllPortsSameDT=off  OutDataTypeStr=boolean
  external_fault_latch : Outport  OutDataTypeStr=boolean  PortDimensions=1
  wires:
  ERRI_raw/1 -> Clear_Only_When_Raw_Healthy/2, ERRI_Active_Low/1
  ERRU_raw/1 -> ERRU_Active_Low/1, Clear_Only_When_Raw_Healthy/3
  ERRI_Active_Low/1 -> External_Fault_OR/1
  ERRU_Active_Low/1 -> External_Fault_OR/2
  clear_fault/1 -> Clear_Only_When_Raw_Healthy/1
  [isr_retain_external_fault] -> Retained_External_Fault/2
  [isr_raw_external_fault] -> External_Fault_Latch_OR/1
  [isr_external_fault_previous] -> Retained_External_Fault/1
  Retained_External_Fault/1 -> External_Fault_Latch_OR/2
  Retain_Unless_Safe_Clear/1 -> [isr_retain_external_fault]
  External_Fault_Latch_Z/1 -> [isr_external_fault_previous]
  Clear_Only_When_Raw_Healthy/1 -> Retain_Unless_Safe_Clear/1
  External_Fault_Latch_OR/1 -> external_fault_latch/1, External_Fault_Latch_Z/1
  External_Fault_OR/1 -> [isr_raw_external_fault]

== system AXU5EV_Motor_Control_System/Motor_Control_ISR/Qualified_Runtime/Alignment_Task ==
  note: 对齐使能、启动、复位与输出
  Alignment_Enable : Inport
  Init_Start : Inport  Port=2
  Init_Reset : Inport  Port=3
  travel_fault_latch : Inport  Port=4
  x_mm : Inport  Port=5
  Alignment_Permit : Inport  Port=6  OutDataTypeStr=boolean
  Enabled_Original_MIL : Subsystem
  Software_Alignment_Permit : Logic  AllPortsSameDT=off  OutDataTypeStr=boolean
  Init_Done : Outport
  Init_State_Num : Outport  Port=2
  id_init_ref : Outport  Port=3
  Angle_Init_EN : Outport  Port=4
  Theta_Offset_auto : Outport  Port=5
  x_align_mm_latch : Outport  Port=6
  wires:
  Software_Alignment_Permit/1 -> Enabled_Original_MIL/5(Alignment_Permit)
  Alignment_Permit/1 -> Software_Alignment_Permit/2
  Alignment_Enable/1 -> Software_Alignment_Permit/1
  Enabled_Original_MIL/2(Init_State_Num) -> Init_State_Num/1
  Init_Start/1 -> Enabled_Original_MIL/1(Init_Start)
  Enabled_Original_MIL/3(id_init_ref) -> id_init_ref/1
  Init_Reset/1 -> Enabled_Original_MIL/2(Init_Reset)
  travel_fault_latch/1 -> Enabled_Original_MIL/3(travel_fault_latch)
  x_mm/1 -> Enabled_Original_MIL/4(x_mm)
  Enabled_Original_MIL/1(Init_Done) -> Init_Done/1
  Enabled_Original_MIL/4(Angle_Init_EN) -> Angle_Init_EN/1
  Enabled_Original_MIL/5(Theta_Offset_auto) -> Theta_Offset_auto/1
  Enabled_Original_MIL/6(x_align_mm_latch) -> x_align_mm_latch/1
